simulink library "lib_InverseKinematicsMacroRobotVelocity"  (R2023b)
settings: Solver=VariableStepAuto  StartTime=0.0  StopTime=10.0  RelTol=1e-3
undefined symbols (not defined in the file or in its folder): ikDebugDataStruct, robotParameters, TsControl
settings Model: Creator=murali  LastModifiedBy=BIROMED
settings SolverCC: AlgebraicLoopSolver=TrustRegion
settings DataIOCC: ReturnWorkspaceOutputs=off
settings DebuggingCC: UnconnectedInputMsg=warning  UnconnectedOutputMsg=warning  UnconnectedLineMsg=warning  ArithmeticOperatorsInVariantConditions=warning
settings ModelReferenceCC: EnableRefExpFcnMdlSchedulingChecks=on
settings SFSimCC: SimUseLocalCustomCode=off  CustomCodeUndefinedFunction=UseInterfaceOnly
settings RTWCC: RTWUseLocalCustomCode=off

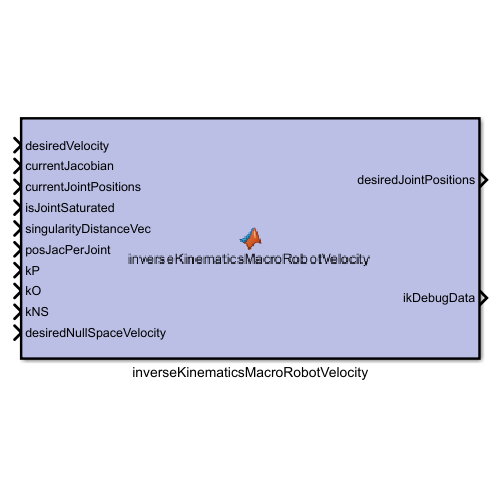
[thumbnail: Simulink's stored preview of the top-level diagram]
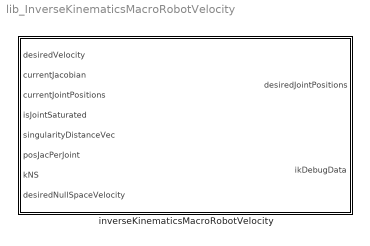
== system lib_InverseKinematicsMacroRobotVelocity ==
  inverseKinematicsMacroRobotVelocity : MATLAB Function  TreatAsAtomicUnit=on

== matlab function lib_InverseKinematicsMacroRobotVelocity/inverseKinematicsMacroRobotVelocity ==
  data: desiredVelocity input double size=[6 1]; currentJacobian input size=[6, nJointsKuka]; currentJointPositions input size=[nJointsKuka 1]; isJointSaturated input double size=[nJointsKuka 1]; singularityDistanceVec input double size=[3 1]; posJacPerJoint input; kNS input double size=1; desiredNullSpaceVelocity input double size=[nJointsKuka 1]; desiredJointPositions output double size=[nJointsKuka 1]; robotParameters parameter Bus: RobotParams; TsControl parameter double size=1; ikDebugData output Bus: IK_DebugData size=1; ikDebugDataStruct parameter Bus: IK_DebugData
%#codegen
function [desiredJointPositions, ikDebugData]   = inverseKinematicsMacroRobotVelocity(desiredVelocity, currentJacobian, currentJointPositions, isJointSaturated, singularityDistanceVec, posJacPerJoint, kNS, desiredNullSpaceVelocity, robotParameters, TsControl, ikDebugDataStruct)

% This just calls the function fun_InverseKinematicsMacroRobotVelocity.m, which has
% the actual code to find the solutions.

[desiredJointPositions, ikDebugData] = fun_InverseKinematicsMacroRobotVelocity(desiredVelocity, currentJacobian, currentJointPositions, isJointSaturated, singularityDistanceVec, posJacPerJoint, kNS, desiredNullSpaceVelocity, robotParameters, TsControl,  ikDebugDataStruct);

end
